simulink model "PO_boost"  (R2023b)
settings: Solver=VariableStepAuto  StartTime=0.0  StopTime=15  RelTol=1e-3
undefined symbols (not defined in the file): sigbuilder_block
libraries: spsSeriesRLCBranchLib x4, SignalEditorBlockLib x3, spsVoltageMeasurementLib x2, spsCurrentMeasurementLib x1, spsDiodeLib x1, spsIGBTDiodeLib x1, spsPVArrayLib x1, spsPWMGeneratorDCDCLib x1, spspowerguiLib x1
settings Model: Creator=B-ONE  LastModifiedBy=happybarsola7gmail.com
settings SolverCC: AlgebraicLoopSolver=TrustRegion
settings OptimizationCC: LifeSpan=inf
settings DebuggingCC: ArithmeticOperatorsInVariantConditions=warning
settings SFSimCC: CustomCodeUndefinedFunction=UseInterfaceOnly
settings CodeAppCC: StateflowObjectComments=on

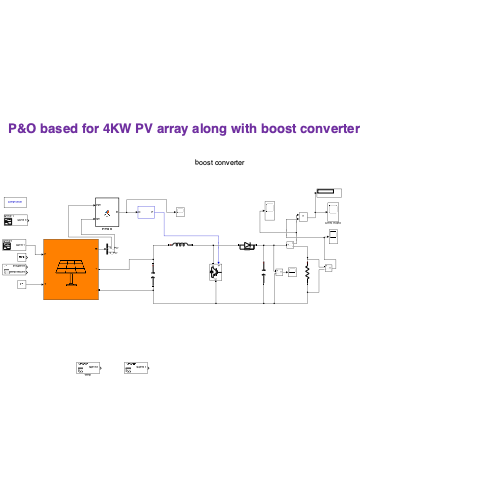
[thumbnail: Simulink's stored preview of the top-level diagram]
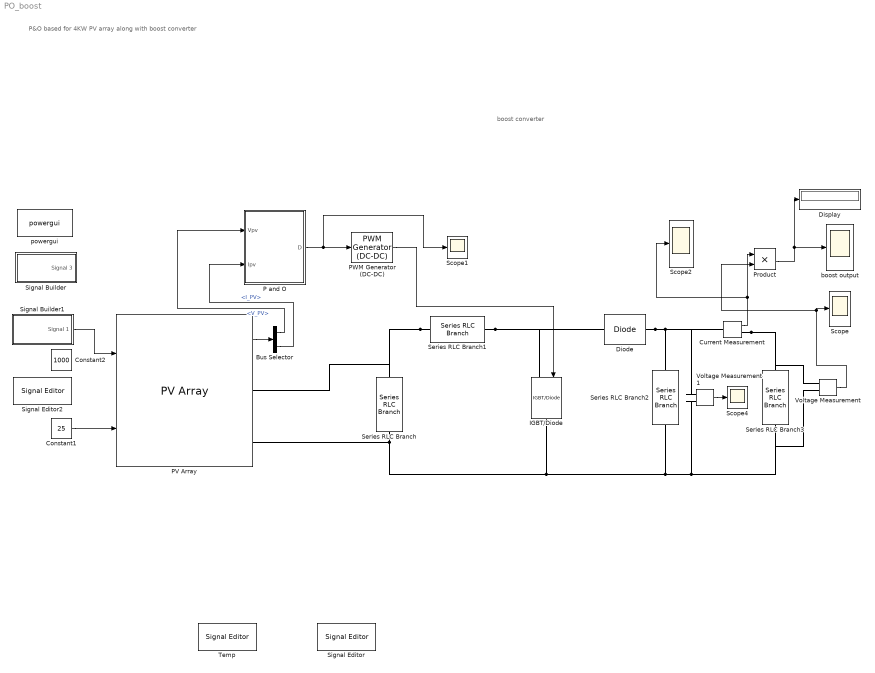
== system PO_boost ==
  note: boost converter
  note: P&O based for 4KW PV array along with boost converter
  Bus Selector : BusSelector  OutputSignals=V_PV,I_PV
  Constant1 : Constant  Value=25
  Constant2 : Constant  Value=1000
  Current Measurement : spsCurrentMeasurementLib/Current Measurement  PhasorSimulation=off  OutputType=Complex  PSBequivalent=0
  Diode : spsDiodeLib/Diode  Ron=0.001  Lon=0  Vf=0.8  IC=0  UseSnubber=0  Rs=500  Cs=250e-9  Measurements=off
  Display : Display
  IGBT/Diode : spsIGBTDiodeLib/IGBT//Diode  Ron=1e-3  Rs=1e5  Cs=inf  Measurements=off
  P and O : MATLAB Function  TreatAsAtomicUnit=on
  PV Array : spsPVArrayLib/PV Array  Npar=4  Nser=4  PlotType=array @ 25 deg.C & specified irradiances  S_vec="[ 1000  500  100 ]"  Temp_C_vec="[ 45 25  ]"  ModuleName=User-defined  PlotWhenSelected=off  Pm=250.205  Ncell=60  Voc=37.3  Isc=8.66  Vm=30.7  Im=8.15  beta_Voc_pc=-0.36901  alpha_Isc_pc=0.086998  beta_Voc=-0.13764  alpha_Isc=0.007534  IL=8.7062  I0=4.1579e-10  nI=1.0189  Rsh=240.6015  Rs=0.23732  RobustModel=off  RobustCellTemperature=313.3991  BAL=on  Tc=1e-6  Tfilter=5e-5
  PWM Generator (DC-DC) : spsPWMGeneratorDCDCLib/PWM Generator (DC-DC)  Fsw=25e3  Ts=0
  Product : Product
  Scope{,1..2,4} (4 alike) : Scope
  Series RLC Branch : spsSeriesRLCBranchLib/Series RLC Branch  LConnTagsString=__new0  RConnTagsString=__new0  BranchType=C  Resistance=1  Inductance=1e-3  SetiL0=off  InitialCurrent=0  Capacitance=0.013  Setx0=off  InitialVoltage=0  Measurements=None
  Series RLC Branch1 : spsSeriesRLCBranchLib/Series RLC Branch  LConnTagsString=__new0  RConnTagsString=__new0  BranchType=L  Resistance=1  Inductance=0.0182  SetiL0=off  InitialCurrent=0  Capacitance=1e-6  Setx0=off  InitialVoltage=0  Measurements=None
  Series RLC Branch2 : spsSeriesRLCBranchLib/Series RLC Branch  LConnTagsString=__new0  RConnTagsString=__new0  BranchType=C  Resistance=1  Inductance=1e-3  SetiL0=off  InitialCurrent=0  Capacitance=0.013  Setx0=off  InitialVoltage=0  Measurements=None
  Series RLC Branch3 : spsSeriesRLCBranchLib/Series RLC Branch  LConnTagsString=__new0  RConnTagsString=__new0  BranchType=R  Resistance=9.2025  Inductance=1e-3  SetiL0=off  InitialCurrent=0  Capacitance=1e-6  Setx0=off  InitialVoltage=0  Measurements=None
  Signal Builder : Subsystem  Tag=STV Subsys  LoadFcn=sigbuilder_block('load');  StartFcn=sigbuilder_block('start');  StopFcn=sigbuilder_block('stop');  ClipboardFcn=sigbuilder_block('clipboard');  mask(Sigbuilder block){tuvar=[0:10]}
      mask help: Simulink:masks:SigbuilderBlock_MD
      mask init:
      | if ~strcmp(get_param(bdroot(gcbh),'SimulationStatus'),'stopped') tuvar = sigbuilder_block('maskInit'); end
      settings: CopyFcn=sigbuilder_block('copy');  DeleteFcn=sigbuilder_block('delete');  ModelCloseFcn=sigbuilder_block('modelClose');  PreSaveFcn=sigbuilder_block('preSave');  PauseFcn=sigbuilder_block('pause');  ContinueFcn=sigbuilder_block('continue');  NameChangeFcn=sigbuilder_block('namechange');  OpenFcn=sigbuilder_block('open',[404 177 695 485 ]);  CloseFcn=sigbuilder_block('close');
      mask Display: plot(0, 0, 100, 100,[2, 2, 32, 32, 2], [68, 8, 8, 68, 68],[32, 2], [38, 38], [32, 19, 2],[53, 60, 44], [32, 17, 17, 2],[16, 16, 31, 31]);txt = getActiveGroup(gcbh);text(2, 100, txt,'verticalAlignment', 'top');
  Signal Builder1 : Subsystem  Tag=STV Subsys  LoadFcn=sigbuilder_block('load');  StartFcn=sigbuilder_block('start');  StopFcn=sigbuilder_block('stop');  ClipboardFcn=sigbuilder_block('clipboard');  mask(Sigbuilder block){tuvar=[0:10]}
      mask help: Simulink:masks:SigbuilderBlock_MD
      mask init:
      | if ~strcmp(get_param(bdroot(gcbh),'SimulationStatus'),'stopped') tuvar = sigbuilder_block('maskInit'); end
      settings: CopyFcn=sigbuilder_block('copy');  DeleteFcn=sigbuilder_block('delete');  ModelCloseFcn=sigbuilder_block('modelClose');  PreSaveFcn=sigbuilder_block('preSave');  PauseFcn=sigbuilder_block('pause');  ContinueFcn=sigbuilder_block('continue');  NameChangeFcn=sigbuilder_block('namechange');  OpenFcn=sigbuilder_block('open',[404 177 894 485 ]);  CloseFcn=sigbuilder_block('close');
      mask Display: plot(0, 0, 100, 100,[2, 2, 32, 32, 2], [68, 8, 8, 68, 68],[32, 2], [38, 38], [32, 19, 2],[53, 60, 44], [32, 17, 17, 2],[16, 16, 31, 31]);txt = getActiveGroup(gcbh);text(2, 100, txt,'verticalAlignment', 'top');
  Signal Editor : SignalEditorBlockLib/Signal Editor  FileName=GHI.mat  ActiveScenario=Scenario  ActiveSignal=Signal 1  IsBus=off  OutputBusObjectStr=Bus: BusObject  SampleTime=0  Interpolate=off  ZeroCross=off  OutputAfterFinalValue=Setting to zero  Unit=inherit  PreserveSignalName=on  ApplySigPropsToAllScenarios=on  ApplySigPropsToAllSignals=off
  Signal Editor2 : SignalEditorBlockLib/Signal Editor  FileName=GHIandTempScenario.mat  ActiveScenario=ds  ActiveSignal=Irradiance  IsBus=off  OutputBusObjectStr=Bus: BusObject  SampleTime=0  Interpolate=off  ZeroCross=off  OutputAfterFinalValue=Setting to zero  Unit=inherit  PreserveSignalName=on  ApplySigPropsToAllScenarios=on  ApplySigPropsToAllSignals=off
  Temp : SignalEditorBlockLib/Signal Editor  FileName=temp.mat  ActiveScenario=Scenario  ActiveSignal=Signal 1  IsBus=off  OutputBusObjectStr=Bus: BusObject  SampleTime=0  Interpolate=off  ZeroCross=off  OutputAfterFinalValue=Setting to zero  Unit=inherit  PreserveSignalName=on  ApplySigPropsToAllScenarios=on  ApplySigPropsToAllSignals=off
  Voltage Measurement : spsVoltageMeasurementLib/Voltage Measurement  PhasorSimulation=off  OutputType=Complex  PSBequivalent=0
  Voltage Measurement1 : spsVoltageMeasurementLib/Voltage Measurement  PhasorSimulation=off  OutputType=Complex  PSBequivalent=0
  boost output : Scope
  powergui : spspowerguiLib/powergui  Priority=1  SimulationMode=Continuous  SampleTime=50e-6  frequency=60  Iterations=50  frequencyindice=0  Pbase=100e6  ErrMax=1e-4  UnitsV=kV  UnitsW=MW  buscounter=0  FunctionMessages=off  echomessages=off  EnableUseOfTLC=off  CurrentSourceSwitches=off  DisableSnubberDevices=off  DisableRonSwitches=off  DisableVfSwitches=off  DisplayEquations=off  AutomaticDiscreteSolvers=off  SolverType=Tustin/Backward Euler (TBE)  Interpol=off  ExternalGateDelay=off  methode=off  Ts=100  x0status=blocks  SPID=on  SwTol=0  HookPort=off  NonlinearTolerance=0  nMaxIteration=15  ContinueOnMaxIteration=off  RestoreLinks=warning  ResistiveCurrentMeasurement=off  Frange=[0:2:500]  Ylog=off  Xlog=on  ShowGrid=off  save=off  variable=ZData  structure=0  ZoomFFT=off  StartTime=0.0  cycles=1  DisplayStyle=1  fundamental=60  FreqAxis=off  MaxFrequency=1000  frequencyindicesteady=1  RmsSteady=1  display=off
  wires:
  PV Array/1 -> Bus Selector/1
  P and O/1(D) -> Scope1/1, PWM Generator (DC-DC)/1
  Product/1 -> boost output/1, Display/1
  Voltage Measurement1/1 -> Scope4/1
  Current Measurement/1 -> Scope2/1, Product/1
  Voltage Measurement/1 -> Product/2, Scope/1
  Bus Selector/2 -> P and O/2(Ipv)  "<I_PV>"
  PWM Generator (DC-DC)/1 -> IGBT/Diode/1
  Bus Selector/1 -> P and O/1(Vpv)  "<V_PV>"
  Constant1/1 -> PV Array/2
  Signal Builder1/1(Signal 1) -> PV Array/1
  connections:
  Series RLC Branch1/RConn1 -- IGBT/Diode/LConn1 -- Diode/LConn1
  Current Measurement/RConn1 -- Voltage Measurement/LConn1 -- Series RLC Branch3/LConn1
  Series RLC Branch2/RConn1 -- PV Array/RConn2 -- Series RLC Branch/RConn1 -- IGBT/Diode/RConn1 -- Series RLC Branch3/RConn1 -- Voltage Measurement/LConn2 -- Voltage Measurement1/LConn2
  Diode/RConn1 -- Current Measurement/LConn1 -- Voltage Measurement1/LConn1 -- Series RLC Branch2/LConn1
  Series RLC Branch1/LConn1 -- Series RLC Branch/LConn1 -- PV Array/RConn1

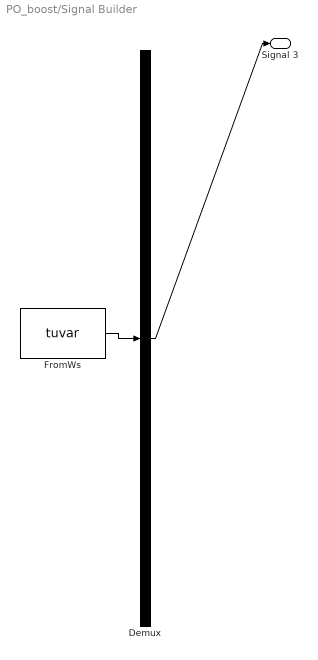
== system PO_boost/Signal Builder ==
  Demux : Demux  Tag=STV Demux  Outputs=1
      settings: DisplayOption=none
  FromWs : FromWorkspace  Tag=STV FromWs  VariableName=tuvar
      SigBuilderData=|
      | common.afterFinalStr = 'Extrapolate'
      | common.sampleTime = 0
      | dataSet.timeRange = [0 10]
      | dataSet.name = 'Group 1'
      | sbobj.Groups.Name = 'Group 1'
      | sbobj.Groups.Signals.Name = 'Signal 3'
      | sbobj.Groups.Signals.XData = [0 3 3 5 5 8 8 10]
      | sbobj.Groups.Signals.YData = [1000 1000 500 500 230 220 805 805]
  Signal 3 : Outport  Tag=STV Outport
  wires:
  FromWs/1 -> Demux/1
  Demux/1 -> Signal 3/1

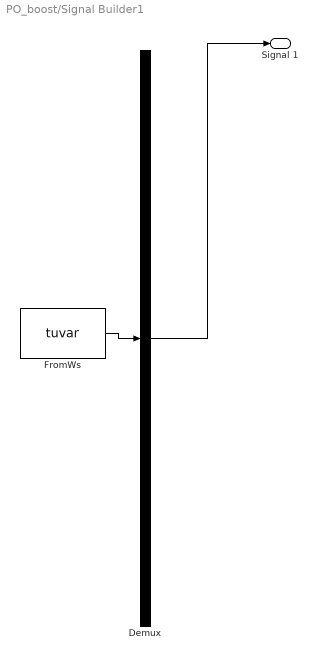
== system PO_boost/Signal Builder1 ==
  Demux : Demux  Tag=STV Demux  Outputs=1
      settings: DisplayOption=none
  FromWs : FromWorkspace  Tag=STV FromWs  VariableName=tuvar
      SigBuilderData=|
      | common.afterFinalStr = 'Extrapolate'
      | common.sampleTime = 0
      | dataSet.timeRange = [0 15]
      | dataSet.name = 'Group 1'
      | sbobj.Groups.Name = 'Group 1'
      | sbobj.Groups.Signals.Name = 'Signal 1'
      | sbobj.Groups.Signals.XData = [0 3 3 5 5 8 8 13 13 15]
      | sbobj.Groups.Signals.YData = [1000 1000 405 400 800 800 600 600 1000 1000]
      | sbobj.Groups.TimeRange = [0 15]
  Signal 1 : Outport  Tag=STV Outport
  wires:
  FromWs/1 -> Demux/1
  Demux/1 -> Signal 1/1

== matlab function PO_boost/P and O ==
  settings: updateMethod=DISCRETE  sampleTime=1e-4
  data: Vpv input; D output; Ipv input
function D = P_O(Vpv,Ipv)
 Dmax=0.9;
 Dmin=0.1;
 Dinit=0.9;
 deltaD=1e-4;
 persistent Dpre Ppre Vpre;
 
 %first run
     if isempty(Dpre)
         Dpre=Dinit;
         Vpre=0;
         Ppre=0;
     end
 Ppv=Vpv*Ipv;
 dp=Ppv-Ppre;
 dv=Vpv-Vpre;
 
     if dp~=0 
             if(dp>0)
                     if(dv<0)
                         D=Dpre+deltaD;
                     else
                         D=Dpre-deltaD;
                     end     
             else                   
                     if(dv<0)
                         D=Dpre-deltaD;
                     else
                         D=Dpre+deltaD;
                     end
             end   
    else
          D=Dpre;
    end
    
    if D>=Dmax || D <= Dmin
        D=Dpre;
    end
    
    Ppre=Ppv;
    Vpre=Vpv;
    Dpre=D;
end
